simulink model "sim_model"  (R2022a)
settings: Solver=VariableStepAuto  StartTime=0.0  StopTime=10.0  RelTol=1e-3
settings Model: Creator=Tan_Tram  LastModifiedBy=Tan_Tram

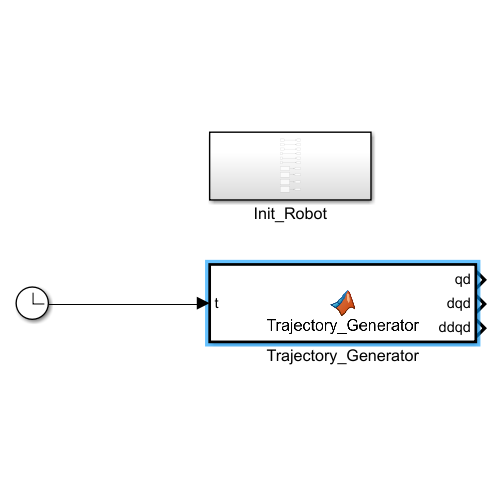
[thumbnail: Simulink's stored preview of the top-level diagram]
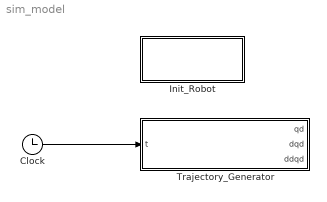
== system sim_model ==
  Clock : Clock
  Init_Robot : Subsystem
  Trajectory_Generator : MATLAB Function  TreatAsAtomicUnit=on
  wires:
  Clock/1 -> Trajectory_Generator/1(t)

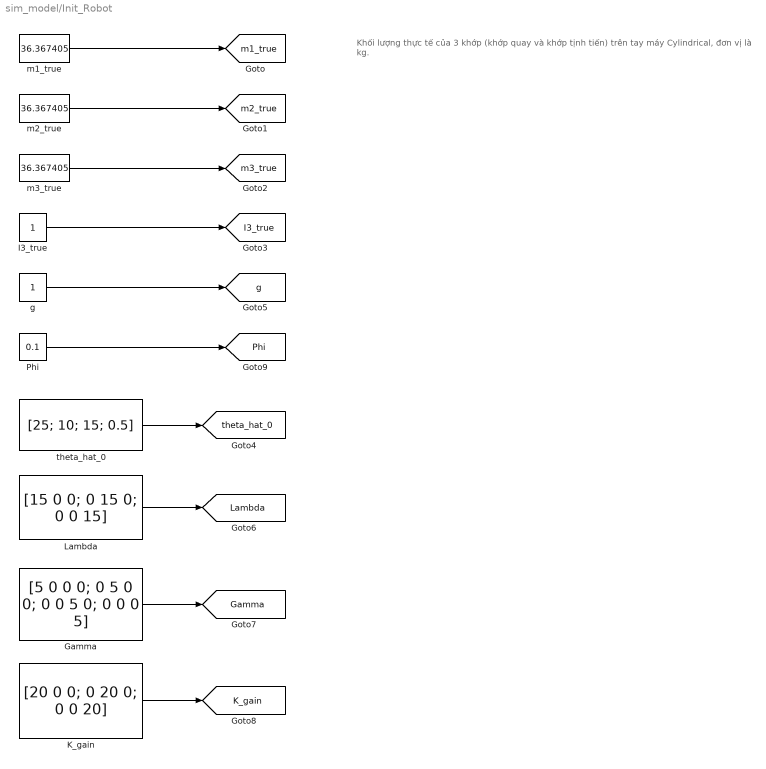
== system sim_model/Init_Robot ==
  note: Khối lượng thực tế của 3 khớp (khớp quay và khớp tịnh tiến) trên tay máy Cylindrical, đơn vị là kg.
  Gamma : Constant  Value=[5 0 0 0; 0 5 0 0; 0 0 5 0; 0 0 0 5]
  I3_true : Constant
  K_gain : Constant  Value=[20 0 0; 0 20 0; 0 0 20]
  Lambda : Constant  Value=[15 0 0; 0 15 0; 0 0 15]
  Phi : Constant  Value=0.1
  g : Constant
  m1_true : Constant  Value=36.367405
  m2_true : Constant  Value=36.367405
  m3_true : Constant  Value=36.367405
  theta_hat_0 : Constant  Value=[25; 10; 15; 0.5]
  tag scope: Gamma=global, I3_true=global, K_gain=global, Lambda=global, Phi=global, g=global, m1_true=global, m2_true=global, m3_true=global, theta_hat_0=global
  wires:
  m1_true/1 -> [m1_true]
  m2_true/1 -> [m2_true]
  m3_true/1 -> [m3_true]
  I3_true/1 -> [I3_true]
  g/1 -> [g]
  theta_hat_0/1 -> [theta_hat_0]
  Lambda/1 -> [Lambda]
  Gamma/1 -> [Gamma]
  Phi/1 -> [Phi]
  K_gain/1 -> [K_gain]

== matlab function sim_model/Trajectory_Generator ==
  data: t input; qd output; dqd output; ddqd output
function [qd, dqd, ddqd] = Trajectory_Generator(t)
    
    A = [1.0; 1.0; 1.0];
    w = [pi; pi; pi];    
    
    qd = A .* sin(w * t);             
    dqd = A .* w .* cos(w * t);      
    ddqd = -A .* (w.^2) .* sin(w * t);
end
